simulink model "IEEE13_coord"  (R2024b)
settings: Solver=ode4  StartTime=0.0  StopTime=1.3  FixedStep=Ts  MaxStep=1e-4  RelTol=1e-4
InitFcn:
  | a=1; % Loading Factor
  | Ts=50e-6;
  | % phase to sequence conversion of RXB matrices
  | c=1*exp(sqrt(-1)*(120*pi/180));
  | T=[1 1 1;1 c*c c;1 c c*c];
  | Tinv=1/3*[1 1 1;1 c c*c;1 c*c c];
  | 
  | % Simulation data for the IEEE 13 Node Test Feeder model
  | mi2km = 1.60934;%  miles to km conversion
  | ft2km = 0.0003048; % feet to km conversion
  | ms2F = 1*1e-6/(2*pi*60);% microsiemens to Farads conversion
  | 
  | 
  | %% Configuration 601
  | % Series Resitance and Reactance - ohm/mile
  | R_601 = [0.3465 0.1560 0.1580;0.1560 0.3375 0.1535;0.1580 0.1535 0.3414];
  | X_601 = [1.1079 0.5017 0.4236;0.5017 1.0478 0.3849;0.4236 0.3849 1.0348];
  | % charging susceptance - microsiemens/mile
  | B_601 = [6.2998 -1.9958 -1.2595;-1.9958 5.9597 -0.7417;-1.2595 -0.7417 5.6386];
  | 
  | R_601 = R_601/mi2km;
  | Rseq=Tinv*R_601*T;
  | R1_601=Rseq(2,2);R0_601=Rseq(1,1);
  | 
  | L_601 = (X_601/(2*pi*60))/mi2km;
  | Lseq=Tinv*L_601*T;
  | L1_601=Lseq(2,2);L0_601=Lseq(1,1);
  | 
  | C_601 =(B_601*ms2F)/mi2km;
  | Cseq=Tinv*C_601*T;
  | C1_601=Cseq(2,2);C0_601=Cseq(1,1);
  | 
  | %% Configuration 602 - series reactance - ohm/mile
  | R_602 = [0.7526 0.1580 0.1560;0.1580 0.7475 0.1535;0.1560 0.1535 0.7436];
  | X_602 = [1.1814 0.4236 0.5017;0.4236 1.1983 0.3849;0.5017 0.3849 1.2112];
  | % charging susceptance - microsiemens/mile
  | B_602 = [5.6990 -1.0817 -1.6905;-1.0817 5.1795 -0.6588;-1.6905 -0.6588 5.4246];
  | 
  | R_602 = R_602/mi2km;
  | Rseq=Tinv*R_602*T;
  | R1_602=Rseq(2,2);R0_602=Rseq(1,1);
  | 
  | L_602 = (X_602/(2*pi*60))/mi2km;
  | Lseq=Tinv*L_602*T;
  | L1_602=Lseq(2,2);L0_602=Lseq(1,1);
  | 
  | C_602 =(B_602*ms2F)/mi2km;
  | Cseq=Tinv*C_602*T;
  | C1_602=Cseq(2,2);C0_602=Cseq(1,1);
  | %% Configuration 603 - series reactance - ohm/mile
  | R_603 = [0 0 0;0 1.3294 0.2066;0 0.2066 1.3238];
  | X_603 = [0 0 0;0 1.3471 0.4591;0 0.4591 1.3569];
  | % charging susceptance - microsiemens/mile
  | B_603 = [0 0 0;0 4.7097 -0.8999;0 -0.8999 4.6658];
  | 
  | % convert for SPS
  | R_603 = R_603/mi2km;
  | Rseq=Tinv*R_603*T;
  | R1_603=Rseq(2,2);R0_603=Rseq(1,1);
  | 
  | ... (+71 lines)
undefined symbols (not defined in the file): find_system
libraries: spsGroundLib x48, spsSeriesRLCBranchLib x46, spsThreePhaseVIMeasurementLib x19, spsControlledVoltageSourceLib x15, spsThreePhaseSeriesRLCLoadLib x7, spsVoltageMeasurementLib x6, spsOnDelayLib x6, spsThreePhasePISectionLineLib x5, spsSeriesRLCLoadLib x5, spsThreePhaseBreakerLib x5, spsMutualInductanceLib x4, spsThreePhaseSeriesRLCBranchLib x4
(part 3 of 3)

== system IEEE13_coord/Regulator 1/Single Phase SVR_B/Voltage Regulator Control/Tap Changer Control ==
  "Up " : Inport
  "Down " : Inport  Port=2
  Constant : Constant  Value=-1
  Constant1 : Constant
  Determine tap position : Subsystem
  Edge Detector : Subsystem  DialogController=POWERSYS.PowerSysDialog  mask(Edge Detector){model=Rising, ic=0}
      mask prompts: model "Edge:"; ic "Input at t = -eps:"
      mask help:
      | This block compares its present input to its previous input.
      |
      | If the input  is a logic signal (TRUE (1) or FALSE (0), the output is a one-step boolean signal TRUE  when  the specified edge (Rising, Falling or Either)  is detected.
      |
      | This block can also be used to detect the slope polarity of a continuous signal. For example, if the specified edge is  "Rising", the output is TRUE as long as the slope of the input signal is positive.
      |
      | The input value at time preceding t=0 is specified by the parameter "Input at t=-eps"
      mask init: same as IEEE13_coord/Regulator 1/Single Phase SVR_A/Voltage Regulator Control/Tap Changer Control/Edge Detector
      mask Help: This block is part of a subset of blocks in the Extras library that does not have documentation associated with it, other than the block mask description.
      mask TypeOptions model: Rising | Falling | Either
      mask Display: plot(0,0,100,100, X1,Y1,X2,Y2,X3,Y3,X4,Y4);
  Logical Operator : Logic  Operator=OR  AllPortsSameDT=off
  Logical Operator1 : Logic  AllPortsSameDT=off
  Mechanical Delay : TransportDelay  DelayTime=MecDelay  InitialOutput=InitialPosition  BufferSize=5120
  Memory : Memory  InitialCondition=1  InheritSampleTime=on
  Relational Operator : RelationalOperator  Operator===  OutDataTypeStr=float('double')  InputSameDT=off
  Switch : Switch  Threshold=0.5  InputSameDT=off
  TapNo : Outport  VectorParamsAs1DForOutWhenUnconnected=off
  Ready : Outport  Port=2  VectorParamsAs1DForOutWhenUnconnected=off
  wires:
  Mechanical Delay/1 -> TapNo/1, Relational Operator/2
  Logical Operator1/1 -> Determine tap position/Trigger
  "Up "/1 -> Logical Operator/1
  "Down "/1 -> Logical Operator/2, Switch/2
  Constant/1 -> Switch/1
  Constant1/1 -> Switch/3
  Switch/1 -> Determine tap position/1(NewTap)
  Determine tap position/1(TapNo) -> Mechanical Delay/1, Relational Operator/1
  Relational Operator/1 -> Memory/1
  Memory/1 -> Logical Operator1/1, Ready/1
  Logical Operator/1 -> Edge Detector/1(In)
  Edge Detector/1(Out) -> Logical Operator1/2

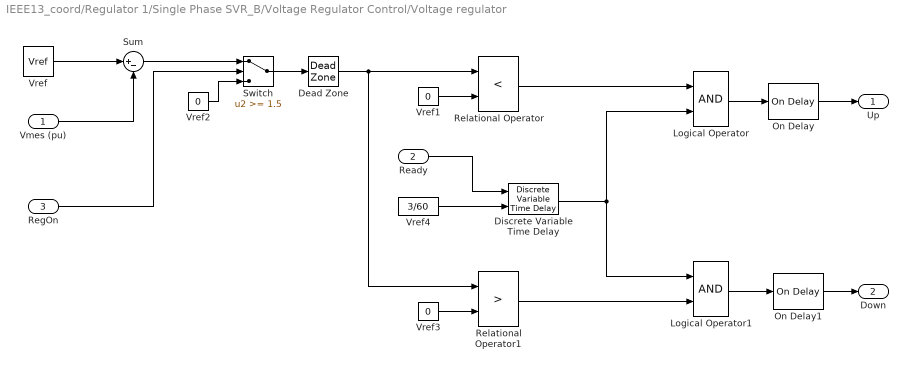
== system IEEE13_coord/Regulator 1/Single Phase SVR_B/Voltage Regulator Control/Voltage regulator ==
  Vmes (pu) : Inport
  Ready : Inport  Port=2
  RegOn : Inport  Port=3
  Dead Zone : DeadZone  LowerValue=-DeadBand/2  UpperValue=+DeadBand/2
  Discrete Variable Time Delay : spsDiscreteVariableTimeDelayLib/Discrete Variable Time Delay  MaxDelay=3/60+Ts  InitialValue=1  Ts=Ts  DFT=on
      settings: LibrarySourceBlock=|
      | sps_lib/Control/Discrete Variable
      | Time Delay
  Logical Operator : Logic  AllPortsSameDT=off
  Logical Operator1 : Logic  AllPortsSameDT=off
  On Delay : spsOnDelayLib/On Delay  DelayType=On delay  delay=TimeDelay  ic=0  Ts=Ts
  On Delay1 : spsOnDelayLib/On Delay  DelayType=On delay  delay=TimeDelay  ic=0  Ts=Ts
  Relational Operator : RelationalOperator  Operator=<  InputSameDT=off
  Relational Operator1 : RelationalOperator  Operator=>  InputSameDT=off
  Sum : Sum  Inputs=|+-  SaturateOnIntegerOverflow=on
  Switch : Switch  Threshold=1.5  InputSameDT=off
  Vref : Constant  Value=Vref
  Vref1 : Constant  Value=0
  Vref2 : Constant  Value=0
  Vref3 : Constant  Value=0
  Vref4 : Constant  Value=3/60
  Up : Outport  VectorParamsAs1DForOutWhenUnconnected=off
  Down : Outport  Port=2  VectorParamsAs1DForOutWhenUnconnected=off
  wires:
  Vref2/1 -> Switch/3
  RegOn/1 -> Switch/2
  Switch/1 -> Dead Zone/1
  Sum/1 -> Switch/1
  Vref/1 -> Sum/1
  Vmes (pu)/1 -> Sum/2
  Dead Zone/1 -> Relational Operator1/1, Relational Operator/1
  Vref1/1 -> Relational Operator/2
  Relational Operator/1 -> Logical Operator/1
  Ready/1 -> Discrete Variable Time Delay/1
  Logical Operator/1 -> On Delay/1
  On Delay/1 -> Up/1
  Relational Operator1/1 -> Logical Operator1/2
  Logical Operator1/1 -> On Delay1/1
  On Delay1/1 -> Down/1
  Vref3/1 -> Relational Operator1/2
  Discrete Variable Time Delay/1 -> Logical Operator1/1, Logical Operator/2
  Vref4/1 -> Discrete Variable Time Delay/2

== system IEEE13_coord/Regulator 1/Single Phase SVR_C/Voltage Regulator Control/Tap Changer Control ==
  "Up " : Inport
  "Down " : Inport  Port=2
  Constant : Constant  Value=-1
  Constant1 : Constant
  Determine tap position : Subsystem
  Edge Detector : Subsystem  DialogController=POWERSYS.PowerSysDialog  mask(Edge Detector){model=Rising, ic=0}
      mask prompts: model "Edge:"; ic "Input at t = -eps:"
      mask help:
      | This block compares its present input to its previous input.
      |
      | If the input  is a logic signal (TRUE (1) or FALSE (0), the output is a one-step boolean signal TRUE  when  the specified edge (Rising, Falling or Either)  is detected.
      |
      | This block can also be used to detect the slope polarity of a continuous signal. For example, if the specified edge is  "Rising", the output is TRUE as long as the slope of the input signal is positive.
      |
      | The input value at time preceding t=0 is specified by the parameter "Input at t=-eps"
      mask init: same as IEEE13_coord/Regulator 1/Single Phase SVR_A/Voltage Regulator Control/Tap Changer Control/Edge Detector
      mask Help: This block is part of a subset of blocks in the Extras library that does not have documentation associated with it, other than the block mask description.
      mask TypeOptions model: Rising | Falling | Either
      mask Display: plot(0,0,100,100, X1,Y1,X2,Y2,X3,Y3,X4,Y4);
  Logical Operator : Logic  Operator=OR  AllPortsSameDT=off
  Logical Operator1 : Logic  AllPortsSameDT=off
  Mechanical Delay : TransportDelay  DelayTime=MecDelay  InitialOutput=InitialPosition  BufferSize=5120
  Memory : Memory  InitialCondition=1  InheritSampleTime=on
  Relational Operator : RelationalOperator  Operator===  OutDataTypeStr=float('double')  InputSameDT=off
  Switch : Switch  Threshold=0.5  InputSameDT=off
  TapNo : Outport  VectorParamsAs1DForOutWhenUnconnected=off
  Ready : Outport  Port=2  VectorParamsAs1DForOutWhenUnconnected=off
  wires:
  Edge Detector/1(Out) -> Logical Operator1/2
  Logical Operator/1 -> Edge Detector/1(In)
  Memory/1 -> Ready/1, Logical Operator1/1
  Relational Operator/1 -> Memory/1
  Determine tap position/1(TapNo) -> Relational Operator/1, Mechanical Delay/1
  Switch/1 -> Determine tap position/1(NewTap)
  Constant1/1 -> Switch/3
  Constant/1 -> Switch/1
  "Down "/1 -> Switch/2, Logical Operator/2
  "Up "/1 -> Logical Operator/1
  Logical Operator1/1 -> Determine tap position/Trigger
  Mechanical Delay/1 -> Relational Operator/2, TapNo/1

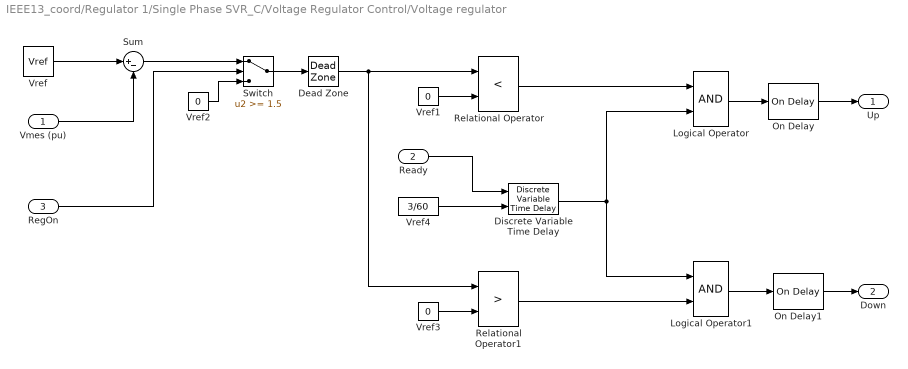
== system IEEE13_coord/Regulator 1/Single Phase SVR_C/Voltage Regulator Control/Voltage regulator ==
  Vmes (pu) : Inport
  Ready : Inport  Port=2
  RegOn : Inport  Port=3
  Dead Zone : DeadZone  LowerValue=-DeadBand/2  UpperValue=+DeadBand/2
  Discrete Variable Time Delay : spsDiscreteVariableTimeDelayLib/Discrete Variable Time Delay  MaxDelay=3/60+Ts  InitialValue=1  Ts=Ts  DFT=on
      settings: LibrarySourceBlock=|
      | sps_lib/Control/Discrete Variable
      | Time Delay
  Logical Operator : Logic  AllPortsSameDT=off
  Logical Operator1 : Logic  AllPortsSameDT=off
  On Delay : spsOnDelayLib/On Delay  DelayType=On delay  delay=TimeDelay  ic=0  Ts=Ts
  On Delay1 : spsOnDelayLib/On Delay  DelayType=On delay  delay=TimeDelay  ic=0  Ts=Ts
  Relational Operator : RelationalOperator  Operator=<  InputSameDT=off
  Relational Operator1 : RelationalOperator  Operator=>  InputSameDT=off
  Sum : Sum  Inputs=|+-  SaturateOnIntegerOverflow=on
  Switch : Switch  Threshold=1.5  InputSameDT=off
  Vref : Constant  Value=Vref
  Vref1 : Constant  Value=0
  Vref2 : Constant  Value=0
  Vref3 : Constant  Value=0
  Vref4 : Constant  Value=3/60
  Up : Outport  VectorParamsAs1DForOutWhenUnconnected=off
  Down : Outport  Port=2  VectorParamsAs1DForOutWhenUnconnected=off
  wires:
  Vref4/1 -> Discrete Variable Time Delay/2
  Discrete Variable Time Delay/1 -> Logical Operator/2, Logical Operator1/1
  Vref3/1 -> Relational Operator1/2
  On Delay1/1 -> Down/1
  Logical Operator1/1 -> On Delay1/1
  Relational Operator1/1 -> Logical Operator1/2
  On Delay/1 -> Up/1
  Logical Operator/1 -> On Delay/1
  Ready/1 -> Discrete Variable Time Delay/1
  Relational Operator/1 -> Logical Operator/1
  Vref1/1 -> Relational Operator/2
  Dead Zone/1 -> Relational Operator/1, Relational Operator1/1
  Vmes (pu)/1 -> Sum/2
  Vref/1 -> Sum/1
  Sum/1 -> Switch/1
  Switch/1 -> Dead Zone/1
  RegOn/1 -> Switch/2
  Vref2/1 -> Switch/3

== system IEEE13_coord/Regulator 1/Single Phase SVR_A/Voltage Regulator Control/Tap Changer Control/Determine tap position ==
  NewTap : Inport
  Trigger : TriggerPort  VariantControl=Variant
  Memory : Memory  InitialCondition=InitialPosition  InheritSampleTime=on
  Saturation : Saturate  UpperLimit=MinMaxTap(2)  LowerLimit=MinMaxTap(1)
  Sum : Sum  Inputs=|++  SaturateOnIntegerOverflow=on
  TapNo : Outport  InitialOutput=InitialPosition  VectorParamsAs1DForOutWhenUnconnected=off
  wires:
  Saturation/1 -> Memory/1, TapNo/1
  Memory/1 -> Sum/2
  Sum/1 -> Saturation/1
  NewTap/1 -> Sum/1

== system IEEE13_coord/Regulator 1/Single Phase SVR_A/Voltage Regulator Control/Tap Changer Control/Edge Detector ==
  note: Edge or Slope Detector
  In : Inport
  Constant1 : Constant  Value=model
  Demux : Demux  Outputs=2
      settings: DisplayOption=none
  Logical Operator1 : Logic  Operator=OR
  Memory : Memory  InitialCondition=ic  LinearizeAsDelay=on
  Multiport Switch : MultiPortSwitch  InputSameDT=off
  NEGATIVE Edge : Subsystem  TreatAsAtomicUnit=on
  POSITIVE Edge : Subsystem  TreatAsAtomicUnit=on
  either edge : Constant  Value=[1 1]
  neg. edge : Constant  Value=[0 1]
  pos. edge : Constant  Value=[1 0]
  Out : Outport  VectorParamsAs1DForOutWhenUnconnected=off
  wires:
  Logical Operator1/1 -> Out/1
  NEGATIVE Edge/1(OUT) -> Logical Operator1/2
  POSITIVE Edge/1(OUT) -> Logical Operator1/1
  Memory/1 -> POSITIVE Edge/2(IN previous), NEGATIVE Edge/2(IN previous)
  In/1 -> POSITIVE Edge/1(IN), NEGATIVE Edge/1(IN), Memory/1
  pos. edge/1 -> Multiport Switch/2
  neg. edge/1 -> Multiport Switch/3
  Constant1/1 -> Multiport Switch/1
  Multiport Switch/1 -> Demux/1
  Demux/1 -> POSITIVE Edge/Enable
  Demux/2 -> NEGATIVE Edge/Enable
  either edge/1 -> Multiport Switch/4

== system IEEE13_coord/Regulator 1/Single Phase SVR_B/Voltage Regulator Control/Tap Changer Control/Determine tap position ==
  NewTap : Inport
  Trigger : TriggerPort  VariantControl=Variant
  Memory : Memory  InitialCondition=InitialPosition  InheritSampleTime=on
  Saturation : Saturate  UpperLimit=MinMaxTap(2)  LowerLimit=MinMaxTap(1)
  Sum : Sum  Inputs=|++  SaturateOnIntegerOverflow=on
  TapNo : Outport  InitialOutput=InitialPosition  VectorParamsAs1DForOutWhenUnconnected=off
  wires:
  NewTap/1 -> Sum/1
  Sum/1 -> Saturation/1
  Memory/1 -> Sum/2
  Saturation/1 -> TapNo/1, Memory/1

== system IEEE13_coord/Regulator 1/Single Phase SVR_B/Voltage Regulator Control/Tap Changer Control/Edge Detector ==
  note: Edge or Slope Detector
  In : Inport
  Constant1 : Constant  Value=model
  Demux : Demux  Outputs=2
      settings: DisplayOption=none
  Logical Operator1 : Logic  Operator=OR
  Memory : Memory  InitialCondition=ic  LinearizeAsDelay=on
  Multiport Switch : MultiPortSwitch  InputSameDT=off
  NEGATIVE Edge : Subsystem  TreatAsAtomicUnit=on
  POSITIVE Edge : Subsystem  TreatAsAtomicUnit=on
  either edge : Constant  Value=[1 1]
  neg. edge : Constant  Value=[0 1]
  pos. edge : Constant  Value=[1 0]
  Out : Outport  VectorParamsAs1DForOutWhenUnconnected=off
  wires:
  either edge/1 -> Multiport Switch/4
  Demux/2 -> NEGATIVE Edge/Enable
  Demux/1 -> POSITIVE Edge/Enable
  Multiport Switch/1 -> Demux/1
  Constant1/1 -> Multiport Switch/1
  neg. edge/1 -> Multiport Switch/3
  pos. edge/1 -> Multiport Switch/2
  In/1 -> Memory/1, NEGATIVE Edge/1(IN), POSITIVE Edge/1(IN)
  Memory/1 -> NEGATIVE Edge/2(IN previous), POSITIVE Edge/2(IN previous)
  POSITIVE Edge/1(OUT) -> Logical Operator1/1
  NEGATIVE Edge/1(OUT) -> Logical Operator1/2
  Logical Operator1/1 -> Out/1

== system IEEE13_coord/Regulator 1/Single Phase SVR_C/Voltage Regulator Control/Tap Changer Control/Determine tap position ==
  NewTap : Inport
  Trigger : TriggerPort  VariantControl=Variant
  Memory : Memory  InitialCondition=InitialPosition  InheritSampleTime=on
  Saturation : Saturate  UpperLimit=MinMaxTap(2)  LowerLimit=MinMaxTap(1)
  Sum : Sum  Inputs=|++  SaturateOnIntegerOverflow=on
  TapNo : Outport  InitialOutput=InitialPosition  VectorParamsAs1DForOutWhenUnconnected=off
  wires:
  Saturation/1 -> Memory/1, TapNo/1
  Memory/1 -> Sum/2
  Sum/1 -> Saturation/1
  NewTap/1 -> Sum/1

== system IEEE13_coord/Regulator 1/Single Phase SVR_C/Voltage Regulator Control/Tap Changer Control/Edge Detector ==
  note: Edge or Slope Detector
  In : Inport
  Constant1 : Constant  Value=model
  Demux : Demux  Outputs=2
      settings: DisplayOption=none
  Logical Operator1 : Logic  Operator=OR
  Memory : Memory  InitialCondition=ic  LinearizeAsDelay=on
  Multiport Switch : MultiPortSwitch  InputSameDT=off
  NEGATIVE Edge : Subsystem  TreatAsAtomicUnit=on
  POSITIVE Edge : Subsystem  TreatAsAtomicUnit=on
  either edge : Constant  Value=[1 1]
  neg. edge : Constant  Value=[0 1]
  pos. edge : Constant  Value=[1 0]
  Out : Outport  VectorParamsAs1DForOutWhenUnconnected=off
  wires:
  Logical Operator1/1 -> Out/1
  NEGATIVE Edge/1(OUT) -> Logical Operator1/2
  POSITIVE Edge/1(OUT) -> Logical Operator1/1
  Memory/1 -> POSITIVE Edge/2(IN previous), NEGATIVE Edge/2(IN previous)
  In/1 -> POSITIVE Edge/1(IN), NEGATIVE Edge/1(IN), Memory/1
  pos. edge/1 -> Multiport Switch/2
  neg. edge/1 -> Multiport Switch/3
  Constant1/1 -> Multiport Switch/1
  Multiport Switch/1 -> Demux/1
  Demux/1 -> POSITIVE Edge/Enable
  Demux/2 -> NEGATIVE Edge/Enable
  either edge/1 -> Multiport Switch/4

== system IEEE13_coord/Regulator 1/Single Phase SVR_A/Voltage Regulator Control/Tap Changer Control/Edge Detector/NEGATIVE Edge ==
  IN : Inport
  IN previous : Inport  Port=2
  Enable : EnablePort  PropagateVarSize=During execution
  Relational Operator1 : RelationalOperator  Operator=>
  OUT : Outport  VectorParamsAs1DForOutWhenUnconnected=off
  wires:
  Relational Operator1/1 -> OUT/1
  IN previous/1 -> Relational Operator1/1
  IN/1 -> Relational Operator1/2

== system IEEE13_coord/Regulator 1/Single Phase SVR_A/Voltage Regulator Control/Tap Changer Control/Edge Detector/POSITIVE Edge ==
  IN : Inport
  IN previous : Inport  Port=2
  Enable : EnablePort  PropagateVarSize=During execution
  Relational Operator1 : RelationalOperator  Operator=>
  OUT : Outport  VectorParamsAs1DForOutWhenUnconnected=off
  wires:
  Relational Operator1/1 -> OUT/1
  IN previous/1 -> Relational Operator1/2
  IN/1 -> Relational Operator1/1

== system IEEE13_coord/Regulator 1/Single Phase SVR_B/Voltage Regulator Control/Tap Changer Control/Edge Detector/NEGATIVE Edge ==
  IN : Inport
  IN previous : Inport  Port=2
  Enable : EnablePort  PropagateVarSize=During execution
  Relational Operator1 : RelationalOperator  Operator=>
  OUT : Outport  VectorParamsAs1DForOutWhenUnconnected=off
  wires:
  IN/1 -> Relational Operator1/2
  IN previous/1 -> Relational Operator1/1
  Relational Operator1/1 -> OUT/1

== system IEEE13_coord/Regulator 1/Single Phase SVR_B/Voltage Regulator Control/Tap Changer Control/Edge Detector/POSITIVE Edge ==
  IN : Inport
  IN previous : Inport  Port=2
  Enable : EnablePort  PropagateVarSize=During execution
  Relational Operator1 : RelationalOperator  Operator=>
  OUT : Outport  VectorParamsAs1DForOutWhenUnconnected=off
  wires:
  IN/1 -> Relational Operator1/1
  IN previous/1 -> Relational Operator1/2
  Relational Operator1/1 -> OUT/1

== system IEEE13_coord/Regulator 1/Single Phase SVR_C/Voltage Regulator Control/Tap Changer Control/Edge Detector/NEGATIVE Edge ==
  IN : Inport
  IN previous : Inport  Port=2
  Enable : EnablePort  PropagateVarSize=During execution
  Relational Operator1 : RelationalOperator  Operator=>
  OUT : Outport  VectorParamsAs1DForOutWhenUnconnected=off
  wires:
  Relational Operator1/1 -> OUT/1
  IN previous/1 -> Relational Operator1/1
  IN/1 -> Relational Operator1/2

== system IEEE13_coord/Regulator 1/Single Phase SVR_C/Voltage Regulator Control/Tap Changer Control/Edge Detector/POSITIVE Edge ==
  IN : Inport
  IN previous : Inport  Port=2
  Enable : EnablePort  PropagateVarSize=During execution
  Relational Operator1 : RelationalOperator  Operator=>
  OUT : Outport  VectorParamsAs1DForOutWhenUnconnected=off
  wires:
  Relational Operator1/1 -> OUT/1
  IN previous/1 -> Relational Operator1/2
  IN/1 -> Relational Operator1/1

== matlab function IEEE13_coord/D-STATCOM/DST Controller ==
  settings: updateMethod=DISCRETE  sampleTime=50e-6
  data: vpcc input; vinv output; iL input; ic input; en input; mode input; g input; dbg output
function [vinv, dbg] = dstatcom_controller(vpcc, iL, ic, en, mode, g)
% D-STATCOM control in the synchronous reference frame with PI regulators.
% The text of this file is copied into the MATLAB Function block of
% IEEE13_dstatcom.slx by build_dstatcom.
%
%   vpcc  phase-to-ground voltage at the point of connection (V)
%   iL    load current (A)
%   ic    D-STATCOM current, positive into the point of connection (A)
%   en    1 = controller active, 0 = track the grid voltage (no current)
%   mode  1 = cancel load reactive power, harmonics and unbalance
%         2 = regulate the voltage magnitude, plus harmonics and unbalance
%   g     [current-loop bandwidth (Hz); KpDc; KiDc; KpV; KiV; Imax (A peak)]
%         hand-tuned baseline: [1500; 1; 15; 5; 500; 850]
%
%   vinv  inverter voltage command for the averaged converter (V)
%   dbg   [Vdc; idRef; iqRef; id; iq; Vd; theta; f]
%
% The converter is an averaged model: no switching, and the DC link is
% represented by its power balance, C*Vdc*dVdc/dt = -Pac.
%#codegen

Ts = 50e-6; w0 = 2*pi*60;
L = 0.2e-3; R = 5e-3; C = 10e-3;          % coupling filter and DC capacitor
VdcRef = 1000;                            % V
Imax = g(6);                              % current limit; 850 A peak is about 500 kVA
Vref = 480*sqrt(2/3);                     % V peak, 1 pu phase voltage
N = 333;                                  % samples in one fundamental cycle

KpI = 2*pi*g(1)*L;  KiI = 2*pi*g(1)*R;    % current loops
KpDc = g(2);        KiDc = g(3);          % DC-link voltage loop, A/V
KpV = g(4);         KiV = g(5);           % AC voltage loop, A/V
KpPll = 178;        KiPll = 15791;        % PLL, 20 Hz bandwidth

persistent theta xPll xId xIq xDc xV vdc buf bsum idx
if isempty(theta)
    theta = atan2((vpcc(2) - vpcc(3))/sqrt(3), (2*vpcc(1) - vpcc(2) - vpcc(3))/3);
    xPll = 0; xId = 0; xIq = 0; xDc = 0; xV = 0; vdc = VdcRef;
    buf = zeros(N, 4); buf(:, 4) = VdcRef;
    bsum = [0; 0; 0; N*VdcRef];
    idx = 1;
end

% Phase-locked loop on the connection-point voltage
[vd, vq] = abc2dq(vpcc, theta);
vmag = max(hypot(vd, vq), 1);
ePll = vq / vmag;
w = w0 + KpPll*ePll + xPll;

[iLd, iLq] = abc2dq(iL, theta);
[icd, icq] = abc2dq(ic, theta);

% One-cycle moving averages: fundamental active and reactive load current,
% voltage magnitude and DC-link voltage
s = [iLd; iLq; vd; vdc];
bsum = bsum + s - buf(idx, :)';
buf(idx, :) = s';
idx = mod(idx, N) + 1;
avg = bsum / N;

if en < 0.5
    vinv = vpcc;
    xId = 0; xIq = 0; xDc = 0; xV = 0;
    idRef = 0; iqRef = 0;
else
    % DC-link voltage PI: active current drawn from the grid
    eDc = VdcRef - avg(4);
    idc = sat(KpDc*eDc + xDc, 0.3*Imax);
    xDc = sat(xDc + KiDc*eDc*Ts, 0.3*Imax);

    idRef = (iLd - avg(1)) - idc;
    if mode < 1.5
        iqRef = iLq;
    else
        % AC voltage PI: negative q current injects reactive power
        eV = Vref - avg(3);
        iqv = sat(KpV*eV + xV, Imax);
        xV = sat(xV + KiV*eV*Ts, Imax);
        iqRef = (iLq - avg(2)) - iqv;
    end
    m = hypot(idRef, iqRef);
    if m > Imax
        idRef = idRef*Imax/m; iqRef = iqRef*Imax/m;
    end

    % Current PI loops with voltage feed-forward and cross-coupling terms
    eD = idRef - icd; eQ = iqRef - icq;
    vdCmd = vd + KpI*eD + xId - w*L*icq;
    vqCmd = vq + KpI*eQ + xIq + w*L*icd;
    vlim = vdc / sqrt(3);
    vm = hypot(vdCmd, vqCmd);
    if vm > vlim
        vdCmd = vdCmd*vlim/vm; vqCmd = vqCmd*vlim/vm;
    else
        xId = xId + KiI*eD*Ts; xIq = xIq + KiI*eQ*Ts;
    end

    % The output reaches the network one sample later: advance the angle
    vinv = dq2abc(vdCmd, vqCmd, theta + 1.5*w*Ts);

    pac = 1.5*(vdCmd*icd + vqCmd*icq);
    vdc = max(vdc - Ts*pac/(C*vdc), 100);
end

dbg = [vdc; idRef; iqRef; icd; icq; vd; theta; w/(2*pi)];

xPll = xPll + KiPll*ePll*Ts;
theta = mod(theta + w*Ts, 2*pi);
end

function [d, q] = abc2dq(x, th)
al = (2*x(1) - x(2) - x(3)) / 3;
be = (x(2) - x(3)) / sqrt(3);
d =  al*cos(th) + be*sin(th);
q = -al*sin(th) + be*cos(th);
end

function x = dq2abc(d, q, th)
al = d*cos(th) - q*sin(th);
be = d*sin(th) + q*cos(th);
x = [al; -al/2 + sqrt(3)/2*be; -al/2 - sqrt(3)/2*be];
end

function y = sat(u, lim)
y = min(max(u, -lim), lim);
end

== matlab function IEEE13_coord/DVR/DVR Controller ==
  settings: updateMethod=DISCRETE  sampleTime=50e-6
  data: vs input; vinj output; vl input; il input; en input; g input; dbg output
function [vinj, dbg] = dvr_controller(vs, vl, il, en, g)
% DVR control: feed-forward of the missing supply voltage plus PI trim of
% the load voltage in the synchronous reference frame.
% The text of this file is copied into the MATLAB Function block of
% IEEE13_dvr.slx by build_dvr.
%
%   vs    supply-side phase-to-ground voltage (V)
%   vl    load-side phase-to-ground voltage (V)
%   il    current through the DVR (A)
%   en    1 = controller active, 0 = inject nothing
%   g     [KpV; KiV; injection limit (pu); load-voltage target during a
%         disturbance (pu); usable battery energy (kJ)]
%         baseline [0.2; 200; 0.5; 1; 1e6]: full restoration, unlimited energy
%
%   vinj  series voltage command for the averaged converter (V)
%   dbg   [Pinj; Einj; trimD; trimQ; vLd; vLq; battery left (0 to 1);
%         flags: 1 = disturbance detected, 2 = battery empty, 3 = both]
%
% The converter is an averaged model with no switching. The battery is an
% energy store: when it is empty the DVR stops injecting.
%#codegen

Ts = 50e-6; w0 = 2*pi*60;
Vref = 480*sqrt(2/3);                     % V peak, 1 pu phase voltage
Vmax = g(3)*Vref;                         % injection limit per phase
N = 333;                                  % samples in one fundamental cycle

KpV = g(1);  KiV = g(2);                  % load-voltage loops
Ecap = g(5)*1e3;                          % usable battery energy, J
KpPll = 44;  KiPll = 987;                 % PLL, 5 Hz bandwidth

persistent theta xPll xD xQ buf bsum idx E Eb hold empty
if isempty(theta)
    theta = atan2((vs(2) - vs(3))/sqrt(3), (2*vs(1) - vs(2) - vs(3))/3);
    xPll = 0; xD = 0; xQ = 0; E = 0;
    Eb = Ecap; hold = 0; empty = 0;
    buf = zeros(N, 1); bsum = 0; idx = 1;
end

% Slow PLL on the supply voltage. The one-cycle average removes the ripple
% from unbalance, so the angle holds its pre-fault phase through a sag.
[vsd, vsq] = abc2dq(vs, theta);
bsum = bsum + vsq - buf(idx);
buf(idx) = vsq;
idx = mod(idx, N) + 1;
ePll = (bsum / N) / Vref;
w = w0 + KpPll*ePll + xPll;

[vld, vlq] = abc2dq(vl, theta);

% Disturbance detection: the supply vector leaves its nominal position by
% more than 0.1 pu. It is held for one cycle so that the ripple of an
% unbalanced fault does not release it.
if hypot(vsd - Vref, vsq) > 0.1*Vref
    hold = N;
elseif hold > 0
    hold = hold - 1;
end
Vtgt = Vref;
if hold > 0, Vtgt = g(4)*Vref; end

if en < 0.5 || empty > 0.5
    vinj = zeros(3, 1);
    xD = 0; xQ = 0; trimD = 0; trimQ = 0;
else
    eD = Vtgt - vld; eQ = -vlq;
    trimD = KpV*eD + xD;
    trimQ = KpV*eQ + xQ;

    % The output reaches the network one sample later: advance the angle.
    % The zero-sequence part of the supply voltage is removed directly.
    v0 = (vs(1) + vs(2) + vs(3)) / 3;
    u = dq2abc(Vtgt - vsd + trimD, -vsq + trimQ, theta + 1.5*w*Ts) - v0;
    vinj = min(max(u, -Vmax), Vmax);
    if all(abs(u) <= Vmax)
        xD = xD + KiV*eD*Ts; xQ = xQ + KiV*eQ*Ts;
    end
end

p = vinj' * il;
E = E + p*Ts;
Eb = min(Eb - p*Ts, Ecap);
if Eb <= 0, empty = 1; end
dbg = [p; E; trimD; trimQ; vld; vlq; max(Eb, 0)/Ecap; (hold > 0) + 2*empty];

xPll = xPll + KiPll*ePll*Ts;
theta = mod(theta + w*Ts, 2*pi);
end

function [d, q] = abc2dq(x, th)
al = (2*x(1) - x(2) - x(3)) / 3;
be = (x(2) - x(3)) / sqrt(3);
d =  al*cos(th) + be*sin(th);
q = -al*sin(th) + be*cos(th);
end

function x = dq2abc(d, q, th)
al = d*cos(th) - q*sin(th);
be = d*sin(th) + q*cos(th);
x = [al; -al/2 + sqrt(3)/2*be; -al/2 - sqrt(3)/2*be];
end

== matlab function IEEE13_coord/PV Plant/PV Controller ==
  settings: updateMethod=DISCRETE  sampleTime=50e-6
  data: vpcc input; vinv output; ig input; res input; en input; kind input; sup input; dbg output
function [vinv, dbg] = dg_controller(vpcc, ig, res, en, kind, sup)
% Averaged model and control of an inverter-interfaced DG plant.
% The text of this file is copied into the MATLAB Function blocks of the
% PV and wind plants by add_dg.
%
%   vpcc  phase-to-ground voltage at the point of connection (V)
%   ig    plant current, positive into the grid (A)
%   res   resource: irradiance in W/m^2 (PV) or wind speed in m/s (wind)
%   en    1 = plant connected, 0 = track the grid voltage (no current)
%   kind  1 = PV plant, 400 kW at 480 V; 2 = wind plant, 500 kW at 4.16 kV
%   sup   0 = unity power factor, stop injecting below 0.5 pu voltage
%         1 = grid support: stay connected and inject reactive current in
%             a sag, 2 pu of current per pu of voltage drop, ahead of active
%             current
%
%   vinv  inverter voltage command for the averaged converter (V)
%   dbg   [Pin_kW; P_kW; Q_kvar; Vdc; id; Vpu; aux; ceased]
%         aux is the DC-voltage reference (PV) or rotor speed in pu (wind)
%
% Source side
%   PV    array I-V curve, perturb-and-observe MPPT on the DC-link voltage
%   wind  full-converter turbine: Cp(lambda) aerodynamics, one-mass rotor,
%         optimal-torque MPPT, ideal power limit at rated, DC chopper
% Grid side (both)
%   PLL, DC-link voltage PI, current PI loops, current limit at 1.1 pu,
%   and the low-voltage behaviour selected by sup.
% There is no switching; the DC link is its power balance.
%#codegen

Ts = 50e-6; w0 = 2*pi*60; N = 333;        % N samples in one cycle
if kind < 1.5
    Vn = 480;  Sr = 450e3; Pr = 400e3; VdcNom = 850;
else
    Vn = 4160; Sr = 550e3; Pr = 500e3; VdcNom = 7500;
end
Vpk  = Vn*sqrt(2/3);                      % 1 pu phase voltage, peak
Imax = 1.1*Sr/(1.5*Vpk);                  % current limit, peak
Zb = Vn^2/Sr; L = 0.1*Zb/w0; R = 0.01*Zb; % coupling filter, as in add_dg
C  = 2*Sr*0.02/VdcNom^2;                  % DC link stores 20 ms of rated power
tRamp = 0.1;                              % soft start, s

KpI = 2*pi*500*L;  KiI = 2*pi*500*R;      % current loops
wdc = 2*pi*20;                            % DC-link voltage loop
KpDc = wdc*C*VdcNom/(1.5*Vpk);  KiDc = KpDc*wdc/4;
KpPll = 178;  KiPll = 15791;              % PLL, 20 Hz bandwidth

% PV array at 25 degC
Voc = 1050; Vmp = 850; Imp = 400e3/Vmp; Isc = 1.07*Imp;
C2 = (Vmp/Voc - 1)/log(1 - Imp/Isc);
C1 = (1 - Imp/Isc)*exp(-Vmp/(C2*Voc));
% Wind turbine. The inertia constant is short so that a wind change shows
% within a simulation of one or two seconds.
vRated = 12; lamOpt = 8.1; cpMax = 0.48; H = 0.5;

persistent theta xPll xId xIq xDc vdc vdcRef buf bsum idx tOn wr ceased chop ...
    pAcc cnt pPrev dirV
if isempty(theta)
    theta = atan2((vpcc(2) - vpcc(3))/sqrt(3), (2*vpcc(1) - vpcc(2) - vpcc(3))/3);
    xPll = 0; xId = 0; xIq = 0; xDc = 0;
    vdc = VdcNom; vdcRef = VdcNom;
    buf = zeros(N, 1); bsum = 0; idx = 1;
    tOn = 0; wr = min(max(res/vRated, 0.3), 1); ceased = 0; chop = 0;
    pAcc = 0; cnt = 0; pPrev = 0; dirV = 1;
end

% Phase-locked loop on the connection-point voltage
[vd, vq] = abc2dq(vpcc, theta);
ePll = vq / max(hypot(vd, vq), 1);
w = w0 + KpPll*ePll + xPll;
[id, iq] = abc2dq(ig, theta);

% One-cycle average of the voltage magnitude for the ride-through logic
bsum = bsum + vd - buf(idx);
buf(idx) = vd;
idx = mod(idx, N) + 1;
vpu = (bsum / N) / Vpk;

% Wind turbine rotor (runs whether or not the plant is connected)
pGen = 0;
if kind > 1.5
    v = max(res, 0) / vRated;
    li = 1/(lamOpt*wr/max(v, 0.05)) - 0.035;
    cp = max(0.5176*(116*li - 5)*exp(-21*li) + 0.0068/(li + 0.035), 0);
    pAero = min(cp/cpMax*v^3, 1);
    tGen = min(wr^2, 1);
    wr = max(wr + Ts*(pAero/wr - tGen)/(2*H), 0.2);
    pGen = tGen*wr*Pr;
end

if en < 0.5
    vinv = vpcc;
    xId = 0; xIq = 0; xDc = 0; vdc = VdcNom; vdcRef = VdcNom; tOn = 0;
    pin = 0; idRef = 0;
else
    tOn = tOn + Ts;
    ramp = min(tOn/tRamp, 1);
    if kind < 1.5
        ipv = max(Isc*max(res, 0)/1000*ramp*(1 - C1*(exp(vdc/(C2*Voc)) - 1)), 0);
        pin = vdc*ipv;
    else
        pin = ramp*pGen;
    end

    % Momentary cessation below 0.5 pu, resume above 0.6 pu; not in support mode
    if sup > 0.5
        ceased = 0;
    elseif vpu < 0.5
        ceased = 1;
    elseif vpu > 0.6
        ceased = 0;
    end

    % Reactive support current (negative q injects reactive power)
    iqRef = 0;
    if sup > 0.5 && vpu < 0.9
        iqRef = -min(2*(1 - vpu), 1) * Imax/1.1;
    end
    idMax = sqrt(max(Imax^2 - iqRef^2, 0));

    % Perturb-and-observe MPPT every two cycles, frozen in abnormal voltage
    if kind < 1.5 && ramp >= 1 && vpu > 0.88
        pAcc = pAcc + pin; cnt = cnt + 1;
        if cnt >= 2*N
            pAvg = pAcc / cnt;
            if pAvg < pPrev, dirV = -dirV; end
            vdcRef = min(max(vdcRef + 3*dirV, 760), 1000);
            pPrev = pAvg; pAcc = 0; cnt = 0;
        end
    end

    % DC-link voltage PI gives the active current, within what is left of
    % the current limit
    if ceased > 0.5
        idRef = 0;
    else
        eDc = vdc - vdcRef;
        u = KpDc*eDc + xDc;
        idRef = min(max(u, 0), idMax);
        if u == idRef, xDc = xDc + KiDc*eDc*Ts; end
    end

    % Current PI loops with voltage feed-forward and cross-coupling terms
    eD = idRef - id; eQ = iqRef - iq;
    vdCmd = vd + KpI*eD + xId - w*L*iq;
    vqCmd = vq + KpI*eQ + xIq + w*L*id;
    vlim = vdc / sqrt(3);
    vm = hypot(vdCmd, vqCmd);
    if vm > vlim
        vdCmd = vdCmd*vlim/vm; vqCmd = vqCmd*vlim/vm;
    else
        xId = xId + KiI*eD*Ts; xIq = xIq + KiI*eQ*Ts;
    end

    % The output reaches the network one sample later: advance the angle
    vinv = dq2abc(vdCmd, vqCmd, theta + 1.5*w*Ts);

    % DC link. The wind plant burns surplus power in a chopper; the PV
    % array limits itself as the voltage rises toward open circuit.
    if kind > 1.5
        if vdc > 1.10*VdcNom, chop = 1; elseif vdc < 1.05*VdcNom, chop = 0; end
        if chop > 0.5, pin = 0; end
    end
    pac = 1.5*(vdCmd*id + vqCmd*iq);
    vdc = max(vdc + Ts*(pin - pac)/(C*vdc), 0.5*VdcNom);
end

if kind < 1.5, aux = vdcRef; else, aux = wr; end
dbg = [pin/1e3; 1.5*(vd*id + vq*iq)/1e3; 1.5*(vq*id - vd*iq)/1e3; ...
    vdc; id; vpu; aux; ceased];

xPll = xPll + KiPll*ePll*Ts;
theta = mod(theta + w*Ts, 2*pi);
end

function [d, q] = abc2dq(x, th)
al = (2*x(1) - x(2) - x(3)) / 3;
be = (x(2) - x(3)) / sqrt(3);
d =  al*cos(th) + be*sin(th);
q = -al*sin(th) + be*cos(th);
end

function x = dq2abc(d, q, th)
al = d*cos(th) - q*sin(th);
be = d*sin(th) + q*cos(th);
x = [al; -al/2 + sqrt(3)/2*be; -al/2 - sqrt(3)/2*be];
end

== matlab function IEEE13_coord/Wind Plant/Wind Controller ==
  settings: updateMethod=DISCRETE  sampleTime=50e-6
  data: vpcc input; vinv output; ig input; res input; en input; kind input; sup input; dbg output
function [vinv, dbg] = dg_controller(vpcc, ig, res, en, kind, sup)
% Averaged model and control of an inverter-interfaced DG plant.
% The text of this file is copied into the MATLAB Function blocks of the
% PV and wind plants by add_dg.
%
%   vpcc  phase-to-ground voltage at the point of connection (V)
%   ig    plant current, positive into the grid (A)
%   res   resource: irradiance in W/m^2 (PV) or wind speed in m/s (wind)
%   en    1 = plant connected, 0 = track the grid voltage (no current)
%   kind  1 = PV plant, 400 kW at 480 V; 2 = wind plant, 500 kW at 4.16 kV
%   sup   0 = unity power factor, stop injecting below 0.5 pu voltage
%         1 = grid support: stay connected and inject reactive current in
%             a sag, 2 pu of current per pu of voltage drop, ahead of active
%             current
%
%   vinv  inverter voltage command for the averaged converter (V)
%   dbg   [Pin_kW; P_kW; Q_kvar; Vdc; id; Vpu; aux; ceased]
%         aux is the DC-voltage reference (PV) or rotor speed in pu (wind)
%
% Source side
%   PV    array I-V curve, perturb-and-observe MPPT on the DC-link voltage
%   wind  full-converter turbine: Cp(lambda) aerodynamics, one-mass rotor,
%         optimal-torque MPPT, ideal power limit at rated, DC chopper
% Grid side (both)
%   PLL, DC-link voltage PI, current PI loops, current limit at 1.1 pu,
%   and the low-voltage behaviour selected by sup.
% There is no switching; the DC link is its power balance.
%#codegen

Ts = 50e-6; w0 = 2*pi*60; N = 333;        % N samples in one cycle
if kind < 1.5
    Vn = 480;  Sr = 450e3; Pr = 400e3; VdcNom = 850;
else
    Vn = 4160; Sr = 550e3; Pr = 500e3; VdcNom = 7500;
end
Vpk  = Vn*sqrt(2/3);                      % 1 pu phase voltage, peak
Imax = 1.1*Sr/(1.5*Vpk);                  % current limit, peak
Zb = Vn^2/Sr; L = 0.1*Zb/w0; R = 0.01*Zb; % coupling filter, as in add_dg
C  = 2*Sr*0.02/VdcNom^2;                  % DC link stores 20 ms of rated power
tRamp = 0.1;                              % soft start, s

KpI = 2*pi*500*L;  KiI = 2*pi*500*R;      % current loops
wdc = 2*pi*20;                            % DC-link voltage loop
KpDc = wdc*C*VdcNom/(1.5*Vpk);  KiDc = KpDc*wdc/4;
KpPll = 178;  KiPll = 15791;              % PLL, 20 Hz bandwidth

% PV array at 25 degC
Voc = 1050; Vmp = 850; Imp = 400e3/Vmp; Isc = 1.07*Imp;
C2 = (Vmp/Voc - 1)/log(1 - Imp/Isc);
C1 = (1 - Imp/Isc)*exp(-Vmp/(C2*Voc));
% Wind turbine. The inertia constant is short so that a wind change shows
% within a simulation of one or two seconds.
vRated = 12; lamOpt = 8.1; cpMax = 0.48; H = 0.5;

persistent theta xPll xId xIq xDc vdc vdcRef buf bsum idx tOn wr ceased chop ...
    pAcc cnt pPrev dirV
if isempty(theta)
    theta = atan2((vpcc(2) - vpcc(3))/sqrt(3), (2*vpcc(1) - vpcc(2) - vpcc(3))/3);
    xPll = 0; xId = 0; xIq = 0; xDc = 0;
    vdc = VdcNom; vdcRef = VdcNom;
    buf = zeros(N, 1); bsum = 0; idx = 1;
    tOn = 0; wr = min(max(res/vRated, 0.3), 1); ceased = 0; chop = 0;
    pAcc = 0; cnt = 0; pPrev = 0; dirV = 1;
end

% Phase-locked loop on the connection-point voltage
[vd, vq] = abc2dq(vpcc, theta);
ePll = vq / max(hypot(vd, vq), 1);
w = w0 + KpPll*ePll + xPll;
[id, iq] = abc2dq(ig, theta);

% One-cycle average of the voltage magnitude for the ride-through logic
bsum = bsum + vd - buf(idx);
buf(idx) = vd;
idx = mod(idx, N) + 1;
vpu = (bsum / N) / Vpk;

% Wind turbine rotor (runs whether or not the plant is connected)
pGen = 0;
if kind > 1.5
    v = max(res, 0) / vRated;
    li = 1/(lamOpt*wr/max(v, 0.05)) - 0.035;
    cp = max(0.5176*(116*li - 5)*exp(-21*li) + 0.0068/(li + 0.035), 0);
    pAero = min(cp/cpMax*v^3, 1);
    tGen = min(wr^2, 1);
    wr = max(wr + Ts*(pAero/wr - tGen)/(2*H), 0.2);
    pGen = tGen*wr*Pr;
end

if en < 0.5
    vinv = vpcc;
    xId = 0; xIq = 0; xDc = 0; vdc = VdcNom; vdcRef = VdcNom; tOn = 0;
    pin = 0; idRef = 0;
else
    tOn = tOn + Ts;
    ramp = min(tOn/tRamp, 1);
    if kind < 1.5
        ipv = max(Isc*max(res, 0)/1000*ramp*(1 - C1*(exp(vdc/(C2*Voc)) - 1)), 0);
        pin = vdc*ipv;
    else
        pin = ramp*pGen;
    end

    % Momentary cessation below 0.5 pu, resume above 0.6 pu; not in support mode
    if sup > 0.5
        ceased = 0;
    elseif vpu < 0.5
        ceased = 1;
    elseif vpu > 0.6
        ceased = 0;
    end

    % Reactive support current (negative q injects reactive power)
    iqRef = 0;
    if sup > 0.5 && vpu < 0.9
        iqRef = -min(2*(1 - vpu), 1) * Imax/1.1;
    end
    idMax = sqrt(max(Imax^2 - iqRef^2, 0));

    % Perturb-and-observe MPPT every two cycles, frozen in abnormal voltage
    if kind < 1.5 && ramp >= 1 && vpu > 0.88
        pAcc = pAcc + pin; cnt = cnt + 1;
        if cnt >= 2*N
            pAvg = pAcc / cnt;
            if pAvg < pPrev, dirV = -dirV; end
            vdcRef = min(max(vdcRef + 3*dirV, 760), 1000);
            pPrev = pAvg; pAcc = 0; cnt = 0;
        end
    end

    % DC-link voltage PI gives the active current, within what is left of
    % the current limit
    if ceased > 0.5
        idRef = 0;
    else
        eDc = vdc - vdcRef;
        u = KpDc*eDc + xDc;
        idRef = min(max(u, 0), idMax);
        if u == idRef, xDc = xDc + KiDc*eDc*Ts; end
    end

    % Current PI loops with voltage feed-forward and cross-coupling terms
    eD = idRef - id; eQ = iqRef - iq;
    vdCmd = vd + KpI*eD + xId - w*L*iq;
    vqCmd = vq + KpI*eQ + xIq + w*L*id;
    vlim = vdc / sqrt(3);
    vm = hypot(vdCmd, vqCmd);
    if vm > vlim
        vdCmd = vdCmd*vlim/vm; vqCmd = vqCmd*vlim/vm;
    else
        xId = xId + KiI*eD*Ts; xIq = xIq + KiI*eQ*Ts;
    end

    % The output reaches the network one sample later: advance the angle
    vinv = dq2abc(vdCmd, vqCmd, theta + 1.5*w*Ts);

    % DC link. The wind plant burns surplus power in a chopper; the PV
    % array limits itself as the voltage rises toward open circuit.
    if kind > 1.5
        if vdc > 1.10*VdcNom, chop = 1; elseif vdc < 1.05*VdcNom, chop = 0; end
        if chop > 0.5, pin = 0; end
    end
    pac = 1.5*(vdCmd*id + vqCmd*iq);
    vdc = max(vdc + Ts*(pin - pac)/(C*vdc), 0.5*VdcNom);
end

if kind < 1.5, aux = vdcRef; else, aux = wr; end
dbg = [pin/1e3; 1.5*(vd*id + vq*iq)/1e3; 1.5*(vq*id - vd*iq)/1e3; ...
    vdc; id; vpu; aux; ceased];

xPll = xPll + KiPll*ePll*Ts;
theta = mod(theta + w*Ts, 2*pi);
end

function [d, q] = abc2dq(x, th)
al = (2*x(1) - x(2) - x(3)) / 3;
be = (x(2) - x(3)) / sqrt(3);
d =  al*cos(th) + be*sin(th);
q = -al*sin(th) + be*cos(th);
end

function x = dq2abc(d, q, th)
al = d*cos(th) - q*sin(th);
be = d*sin(th) + q*cos(th);
x = [al; -al/2 + sqrt(3)/2*be; -al/2 - sqrt(3)/2*be];
end

== matlab function IEEE13_coord/Relay Logic ==
  settings: updateMethod=DISCRETE  sampleTime=50e-6
  data: i650 input; cmd output; t input; cfg input; dbg output
function [cmd, dbg] = fault_relay(i650, t, cfg)
% Fault timing with an inverse-time overcurrent relay at the substation.
% The text of this file is copied into the MATLAB Function block of
% IEEE13_coord.slx by add_relay.
%
%   i650  substation current (A)
%   t     simulation time (s)
%   cfg   [fault start (s); fault location 1 to 3; pickup current (A rms);
%          time multiplier; breaker time (s); backup clearing time (s)]
%
%   cmd   3-by-1 fault command, 1 = fault applied at that location
%   dbg   [largest phase current (A rms); relay progress 0 to 1;
%          trip time (s, -1 before the trip); fault applied]
%
% The fault starts at cfg(1). The relay follows the IEC standard inverse
% curve, t = TMS * 0.14 / ((I/Ip)^0.02 - 1), so a larger fault current is
% cleared sooner. The fault is removed one breaker time after the trip, or
% after the backup time if the current never reaches pickup.
%#codegen

Ts = 50e-6; N = 333;                      % N samples in one cycle

persistent buf bsum idx acc tTrip
if isempty(buf)
    buf = zeros(N, 3); bsum = zeros(1, 3); idx = 1; acc = 0; tTrip = -1;
end

% One-cycle rms of each phase; the relay acts on the largest
sq = (i650(:)').^2;
bsum = bsum + sq - buf(idx, :);
buf(idx, :) = sq;
idx = mod(idx, N) + 1;
I = sqrt(max(max(bsum), 0) / N);

started = t >= cfg(1);
if started && tTrip < 0
    if I > cfg(3)
        acc = acc + Ts*((I/cfg(3))^0.02 - 1) / (0.14*cfg(4));
    else
        acc = 0;
    end
    if acc >= 1 || t >= cfg(1) + cfg(6), tTrip = t; end
end
applied = started && ~(tTrip >= 0 && t >= tTrip + cfg(5));

cmd = zeros(3, 1);
if applied, cmd(min(max(round(cfg(2)), 1), 3)) = 1; end
dbg = [I; min(acc, 1); tTrip; double(applied)];
end
